simulink model "swift_6dof"  (R2026a)
settings: Solver=ode45  StopTime=P.sim.tfinal  MaxStep=0.01  RelTol=1e-6
InitFcn:
  | if ~evalin('base','exist(''P'',''var'')')
  |     evalin('base','swift_placeholder');
  | end
undefined symbols (not defined in the file): P
libraries: aerolibasang x2, aerolibadyn x1, aerolibatmos2 x1
settings Model: Creator=rbilo  LastModifiedBy=Ryan

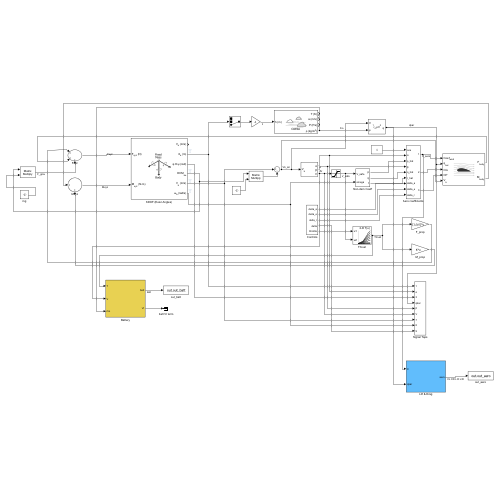
[thumbnail: Simulink's stored preview of the top-level diagram]
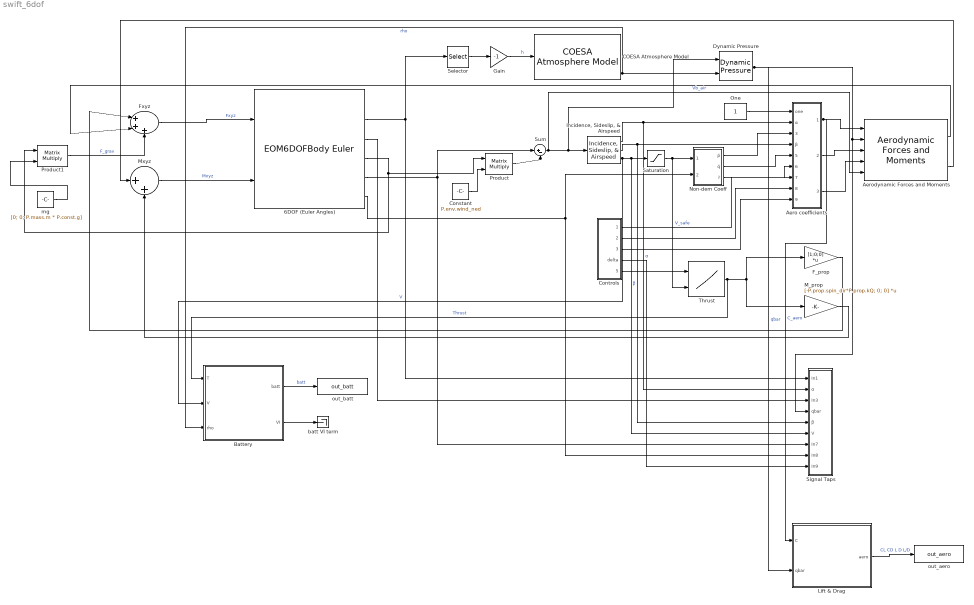
== system swift_6dof ==
  6DOF (Euler Angles) : EOM6DOFBodyEuler  xme_0=P.init.pos0'  Vm_0=P.init.uvw0'  eul_0=P.init.euler0'  pm_0=P.init.om0'  mass_0=P.mass.m  inertia=P.mass.I
  Aero coefficients : Subsystem
  "Aerodynamic Forces and Moments " : aerolibadyn/Aerodynamic Forces and Moments   inputAxes=Wind  outputForceAxes=Body  outputMomentAxes=Body  S=P.geom.S  b=P.geom.b  cbar=P.geom.c
  Battery : Subsystem
  COESA Atmosphere Model : aerolibatmos2/COESA Atmosphere Model  units=Metric (MKS)  spec=1976 COESA-extended U.S. Standard Atmosphere  model=Profile  profile_var=High temperature  profile_percent=1%  profile_alt=5 km (16404 ft)  envelope_var=High temperature  envelope_percent=1%  action=Warning
  Constant : Constant  Value=P.env.wind_ned
  Controls : Subsystem
  Dynamic Pressure : aerolibasang/Dynamic Pressure
  F_prop : Gain  Gain=[1;0;0]  Multiplication=Matrix(K*u)
  Fxyz : Sum  Inputs=|+++
  Gain : Gain  Gain=-1
  "Incidence, Sideslip, & Airspeed" : aerolibasang/Incidence, Sideslip, & Airspeed
  Lift & Drag : Subsystem  Description=L = qbar*S*CL, D = qbar*S*CD, L/D = CL/CD. Output [CL; CD; L; D; L/D]. Added by swift_liftdrag_add.
  M_prop : Gain  Gain=[-P.prop.spin_dir*P.prop.kQ; 0; 0]  Multiplication=Matrix(K*u)
  Mxyz : Sum  Inputs=|++
  Non-dem Coeff : Subsystem
  One : Constant
  Product : Product  Multiplication=Matrix(*)
  Product1 : Product  Multiplication=Matrix(*)
  Saturation : Saturate  UpperLimit=inf  LowerLimit=0.5
  Selector : Selector  InputPortWidth=3  IndexOptions=Index vector (dialog)  Indices=3  OutputSizes=1
  Signal Taps : Subsystem
  Sum : Sum  Inputs=|+-
  Thrust : Lookup_n-D  BreakpointsForDimension1=P.prop.throttle_bp  BreakpointsForDimension2=P.prop.V_bp  Table=P.prop.thrust_map  ExtrapMethod=Clip  InternalRulePriority=Speed  RndMeth=Simplest
      settings: InputPortMap=u0,u1
  batt VI term : Terminator
  mg : Constant  Value=[0; 0; P.mass.m * P.const.g]
  out_aero : ToWorkspace  VariableName=out_aero  SaveFormat=Timeseries  SampleTime=-1
  out_batt : ToWorkspace  VariableName=out_batt  SaveFormat=Timeseries  SampleTime=-1
  wires:
  6DOF (Euler Angles)/2 -> Signal Taps/1(In1), Selector/1
  6DOF (Euler Angles)/4 -> Product1/1, Product/1
  Constant/1 -> Product/2
  Selector/1 -> Gain/1
  Gain/1 -> COESA Atmosphere Model/1  "h"
  Product/1 -> Sum/2
  Sum/1 -> "Incidence, Sideslip, & Airspeed"/1, Dynamic Pressure/1, "Aerodynamic Forces and Moments "/5  "Vb_air"
  "Incidence, Sideslip, & Airspeed"/3 -> Signal Taps/6(V), Saturation/1, Battery/2(V)  "V"
  COESA Atmosphere Model/4 -> Dynamic Pressure/2, Battery/3(rho)  "rho"
  Saturation/1 -> Thrust/2, Non-dem Coeff/1(V_safe)  "V_safe"
  6DOF (Euler Angles)/6 -> Signal Taps/8(In8), Non-dem Coeff/2(omega)
  Dynamic Pressure/1 -> Signal Taps/4(qbar), "Aerodynamic Forces and Moments "/2, Lift & Drag/2(qbar)  "qbar"
  "Incidence, Sideslip, & Airspeed"/1 -> Signal Taps/2(α), Aero coefficients/2(α)  "α"
  "Incidence, Sideslip, & Airspeed"/2 -> Signal Taps/5(β), Aero coefficients/4(β)  "β"
  Aero coefficients/1(Out1) -> "Aerodynamic Forces and Moments "/1, Lift & Drag/1(C)  "C_aero"
  Aero coefficients/2(Out2) -> "Aerodynamic Forces and Moments "/3
  Aero coefficients/3(Out3) -> "Aerodynamic Forces and Moments "/4
  One/1 -> Aero coefficients/1(one)
  Non-dem Coeff/1(p̂) -> Aero coefficients/3(p_hat)
  Non-dem Coeff/2(q̂) -> Aero coefficients/5(q_hat)
  Non-dem Coeff/3(r̂) -> Aero coefficients/6(r_hat)
  Controls/1(delta_a) -> Aero coefficients/7(delta_a)
  Controls/2(delta_e) -> Aero coefficients/8(delta_e)
  Controls/3(delta_r) -> Aero coefficients/9(delta_r)
  Controls/5(throttle) -> Thrust/1
  Thrust/1 -> F_prop/1, M_prop/1, Battery/1(T)  "Thrust"
  mg/1 -> Product1/2
  Product1/1 -> Fxyz/3  "F_grav"
  Fxyz/1 -> 6DOF (Euler Angles)/1  "Fxyz"
  F_prop/1 -> Fxyz/1
  Mxyz/1 -> 6DOF (Euler Angles)/2  "Mxyz"
  M_prop/1 -> Mxyz/2
  "Aerodynamic Forces and Moments "/1 -> Fxyz/2
  "Aerodynamic Forces and Moments "/2 -> Mxyz/1
  6DOF (Euler Angles)/5 -> Signal Taps/7(In7), Sum/1
  6DOF (Euler Angles)/3 -> Signal Taps/3(In3)
  Controls/4(delta) -> Signal Taps/9(In9)
  Battery/1(batt) -> out_batt/1  "batt"
  Battery/2(VI) -> batt VI term/1
  Lift & Drag/1(aero) -> out_aero/1  "CL CD L D L/D"

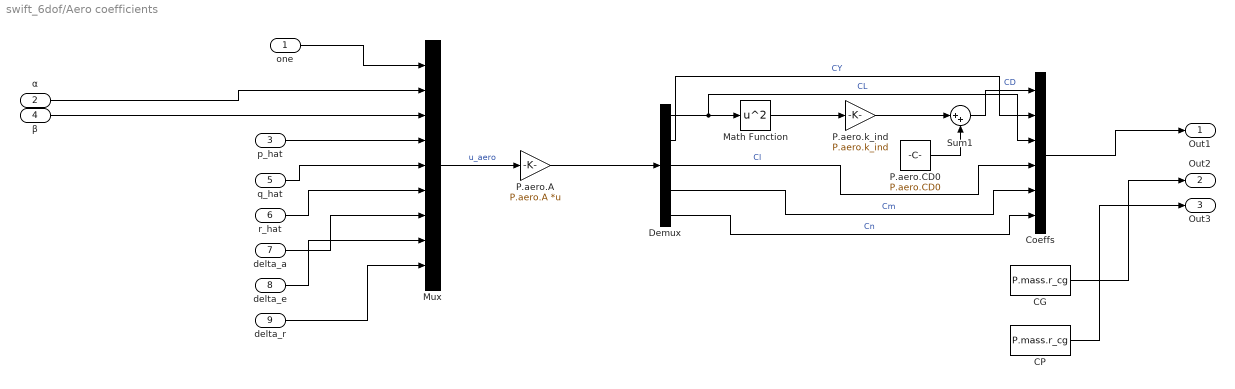
== system swift_6dof/Aero coefficients ==
  one : Inport
  α : Inport  Port=2
  p_hat : Inport  Port=3
  β : Inport  Port=4
  q_hat : Inport  Port=5
  r_hat : Inport  Port=6
  delta_a : Inport  Port=7
  delta_e : Inport  Port=8
  delta_r : Inport  Port=9
  CG : Constant  Value=P.mass.r_cg
  CP : Constant  Value=P.mass.r_cg
  Coeffs : Mux  Inputs=6
  Demux : Demux  Outputs=5
  Math Function : Math  Operator=square
  Mux : Mux  Inputs=9
  P.aero.A : Gain  Gain=P.aero.A  Multiplication=Matrix(K*u)
  P.aero.CD0 : Constant  Value=P.aero.CD0
  P.aero.k_ind : Gain  Gain=P.aero.k_ind
  Sum1 : Sum  Inputs=|++
  Out1 : Outport
  Out2 : Outport  Port=2
  Out3 : Outport  Port=3
  wires:
  P.aero.CD0/1 -> Sum1/2
  p_hat/1 -> Mux/4
  Demux/1 -> Math Function/1, Coeffs/3  "CL"
  delta_r/1 -> Mux/9
  Math Function/1 -> P.aero.k_ind/1
  CP/1 -> Out3/1
  P.aero.k_ind/1 -> Sum1/1
  P.aero.A/1 -> Demux/1
  delta_a/1 -> Mux/7
  Mux/1 -> P.aero.A/1  "u_aero"
  CG/1 -> Out2/1
  Demux/2 -> Coeffs/2  "CY"
  Sum1/1 -> Coeffs/1  "CD"
  β/1 -> Mux/3
  Demux/5 -> Coeffs/6  "Cn"
  Demux/3 -> Coeffs/4  "Cl"
  Demux/4 -> Coeffs/5  "Cm"
  r_hat/1 -> Mux/6
  Coeffs/1 -> Out1/1
  α/1 -> Mux/2
  q_hat/1 -> Mux/5
  one/1 -> Mux/1
  delta_e/1 -> Mux/8

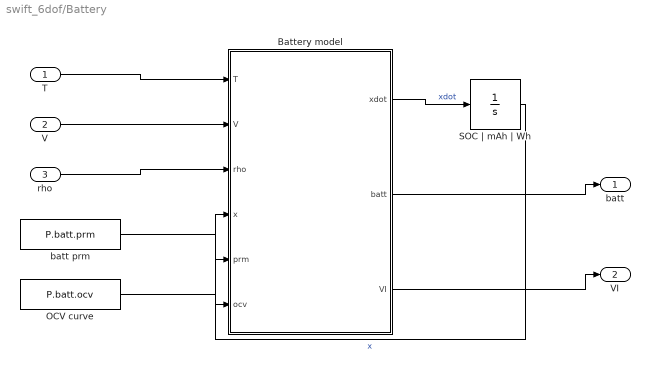
== system swift_6dof/Battery ==
  T : Inport
  V : Inport  Port=2
  rho : Inport  Port=3
  Battery model : MATLAB Function  TreatAsAtomicUnit=on
  OCV curve : Constant  Value=P.batt.ocv
  SOC | mAh | Wh : Integrator  InitialCondition=P.batt.x0  LimitOutput=on  UpperSaturationLimit=[1; inf; inf]  LowerSaturationLimit=[0; 0; 0]
  batt prm : Constant  Value=P.batt.prm
  batt : Outport
  VI : Outport  Port=2
  wires:
  T/1 -> Battery model/1(T)
  V/1 -> Battery model/2(V)
  rho/1 -> Battery model/3(rho)
  SOC | mAh | Wh/1 -> Battery model/4(x)  "x"
  batt prm/1 -> Battery model/5(prm)
  OCV curve/1 -> Battery model/6(ocv)
  Battery model/1(xdot) -> SOC | mAh | Wh/1  "xdot"
  Battery model/2(batt) -> batt/1
  Battery model/3(VI) -> VI/1

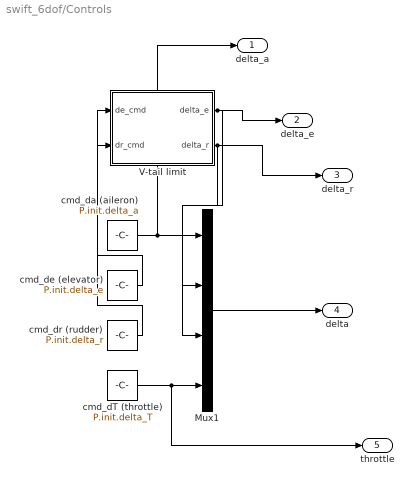
== system swift_6dof/Controls ==
  Mux1 : Mux
  V-tail limit : Subsystem
  cmd_dT (throttle) : Constant  Value=P.init.delta_T
  cmd_da (aileron) : Constant  Value=P.init.delta_a
  cmd_de (elevator) : Constant  Value=P.init.delta_e
  cmd_dr (rudder) : Constant  Value=P.init.delta_r
  delta_a : Outport
  delta_e : Outport  Port=2
  delta_r : Outport  Port=3
  delta : Outport  Port=4
  throttle : Outport  Port=5
  wires:
  Mux1/1 -> delta/1
  cmd_dT (throttle)/1 -> throttle/1, Mux1/4
  cmd_da (aileron)/1 -> delta_a/1, Mux1/1
  cmd_de (elevator)/1 -> V-tail limit/1(de_cmd)
  cmd_dr (rudder)/1 -> V-tail limit/2(dr_cmd)
  V-tail limit/1(delta_e) -> delta_e/1, Mux1/2
  V-tail limit/2(delta_r) -> delta_r/1, Mux1/3

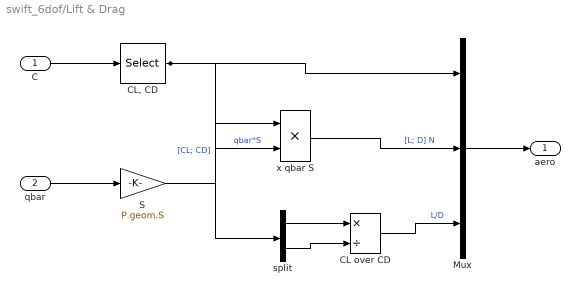
== system swift_6dof/Lift & Drag ==
  C : Inport
  qbar : Inport  Port=2
  CL over CD : Product  Inputs=*/
  "CL, CD" : Selector  InputPortWidth=6  IndexOptions=Index vector (dialog)  Indices=[3 1]  OutputSizes=1
  Mux : Mux  Inputs=3
  S : Gain  Gain=P.geom.S
  split : Demux  Outputs=2
  x qbar S : Product
  aero : Outport
  wires:
  C/1 -> "CL, CD"/1
  qbar/1 -> S/1
  "CL, CD"/1 -> Mux/1, x qbar S/1, split/1  "[CL; CD]"
  S/1 -> x qbar S/2  "qbar*S"
  split/1 -> CL over CD/1
  split/2 -> CL over CD/2
  x qbar S/1 -> Mux/2  "[L; D] N"
  CL over CD/1 -> Mux/3  "L/D"
  Mux/1 -> aero/1

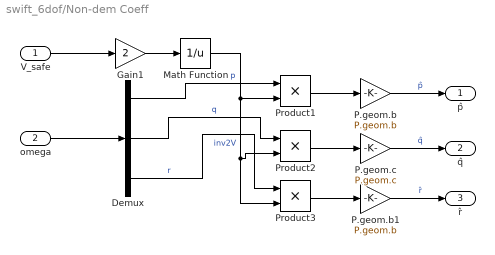
== system swift_6dof/Non-dem Coeff ==
  V_safe : Inport
  omega : Inport  Port=2
  Demux : Demux  Outputs=3
  Gain1 : Gain  Gain=2
  Math Function : Math  Operator=reciprocal
  P.geom.b : Gain  Gain=P.geom.b
  P.geom.b1 : Gain  Gain=P.geom.b
  P.geom.c : Gain  Gain=P.geom.c
  Product1 : Product
  Product2 : Product
  Product3 : Product
  p̂ : Outport
  q̂ : Outport  Port=2
  r̂ : Outport  Port=3
  wires:
  Math Function/1 -> Product2/2, Product3/2, Product1/2  "inv2V"
  Demux/2 -> Product2/1  "q"
  omega/1 -> Demux/1
  Product2/1 -> P.geom.c/1
  Demux/1 -> Product1/1  "p"
  Product1/1 -> P.geom.b/1
  Product3/1 -> P.geom.b1/1
  Gain1/1 -> Math Function/1
  Demux/3 -> Product3/1  "r"
  V_safe/1 -> Gain1/1
  P.geom.c/1 -> q̂/1  "q̂"
  P.geom.b/1 -> p̂/1  "p̂"
  P.geom.b1/1 -> r̂/1  "r̂"

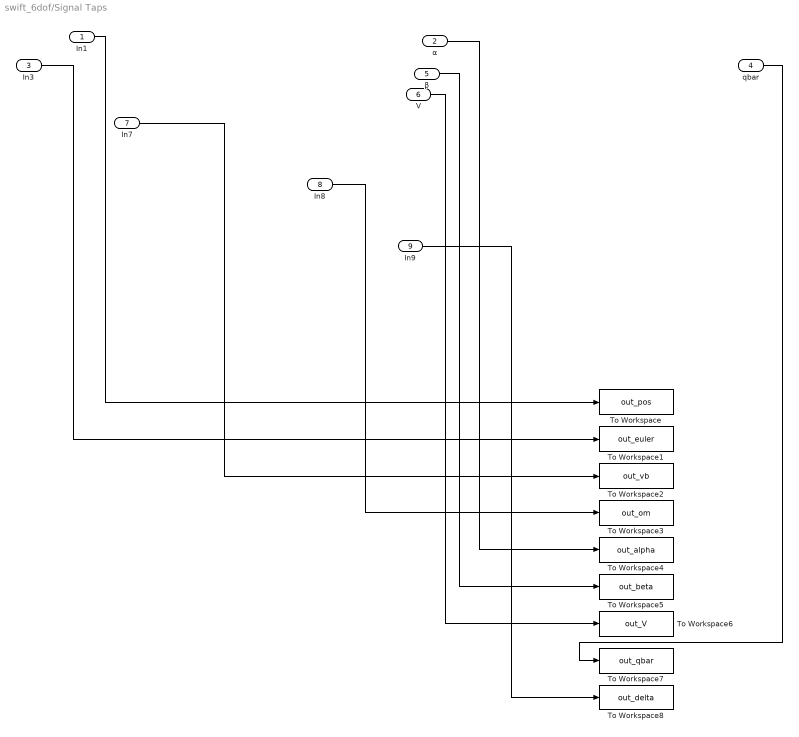
== system swift_6dof/Signal Taps ==
  In1 : Inport
  α : Inport  Port=2
  In3 : Inport  Port=3
  qbar : Inport  Port=4
  β : Inport  Port=5
  V : Inport  Port=6
  In7 : Inport  Port=7
  In8 : Inport  Port=8
  In9 : Inport  Port=9
  To Workspace : ToWorkspace  VariableName=out_pos  SaveFormat=Timeseries  SampleTime=-1
  To Workspace1 : ToWorkspace  VariableName=out_euler  SaveFormat=Timeseries  SampleTime=-1
  To Workspace2 : ToWorkspace  VariableName=out_vb  SaveFormat=Timeseries  SampleTime=-1
  To Workspace3 : ToWorkspace  VariableName=out_om  SaveFormat=Timeseries  SampleTime=-1
  To Workspace4 : ToWorkspace  VariableName=out_alpha  SaveFormat=Timeseries  SampleTime=-1
  To Workspace5 : ToWorkspace  VariableName=out_beta  SaveFormat=Timeseries  SampleTime=-1
  To Workspace6 : ToWorkspace  VariableName=out_V  SaveFormat=Timeseries  SampleTime=-1
  To Workspace7 : ToWorkspace  VariableName=out_qbar  SaveFormat=Timeseries  SampleTime=-1
  To Workspace8 : ToWorkspace  VariableName=out_delta  SaveFormat=Timeseries  SampleTime=-1
  wires:
  V/1 -> To Workspace6/1
  In3/1 -> To Workspace1/1
  α/1 -> To Workspace4/1
  qbar/1 -> To Workspace7/1
  β/1 -> To Workspace5/1
  In7/1 -> To Workspace2/1
  In9/1 -> To Workspace8/1
  In1/1 -> To Workspace/1
  In8/1 -> To Workspace3/1

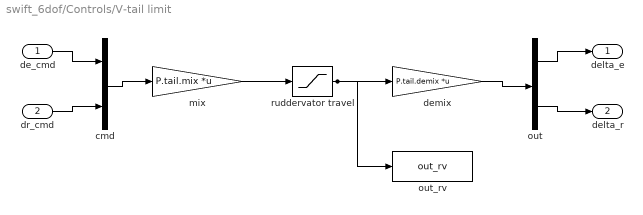
== system swift_6dof/Controls/V-tail limit ==
  de_cmd : Inport
  dr_cmd : Inport  Port=2
  cmd : Mux  Inputs=2
  demix : Gain  Gain=P.tail.demix  Multiplication=Matrix(K*u)
  mix : Gain  Gain=P.tail.mix  Multiplication=Matrix(K*u)
  out : Demux  Outputs=2
  out_rv : ToWorkspace  VariableName=out_rv  SaveFormat=Timeseries  SampleTime=-1
  ruddervator travel : Saturate  UpperLimit=P.tail.drv_max  LowerLimit=-P.tail.drv_max
  delta_e : Outport
  delta_r : Outport  Port=2
  wires:
  de_cmd/1 -> cmd/1
  dr_cmd/1 -> cmd/2
  cmd/1 -> mix/1
  mix/1 -> ruddervator travel/1
  ruddervator travel/1 -> demix/1, out_rv/1
  demix/1 -> out/1
  out/1 -> delta_e/1
  out/2 -> delta_r/1

== matlab function swift_6dof/Battery/Battery model ==
  data: T input; xdot output; V input; rho input; x input; prm input; ocv input; batt output; VI output
function [xdot, batt, VI] = battery(T, V, rho, x, prm, ocv)
%BATTERY  SWIFT battery model. All the physics is in swift_battery_fcn.m.
%   T N, V m/s, rho kg/m^3, x = [SOC; mAh; Wh], prm = P.batt.prm, ocv = P.batt.ocv
[xdot, batt, VI] = swift_battery_fcn(T, V, rho, x, prm, ocv);
